simulink model "Microgrid_RL_Model"  (R2025b)
settings: Solver=ode23tb  StartTime=0.0  StopTime=12.0  MaxStep=0.01  RelTol=1e-8  AbsTol=1e-10
settings Model: Creator=ogare  LastModifiedBy=ogare

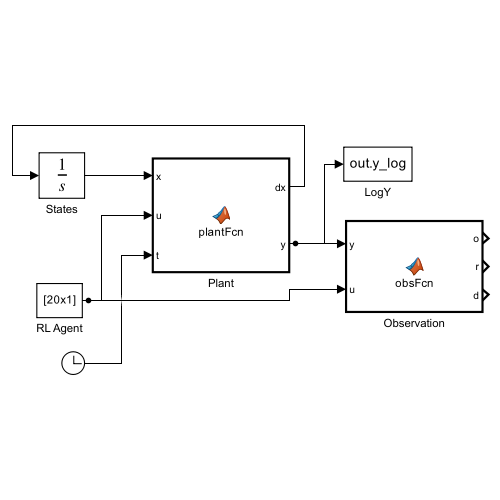
[thumbnail: Simulink's stored preview of the top-level diagram]
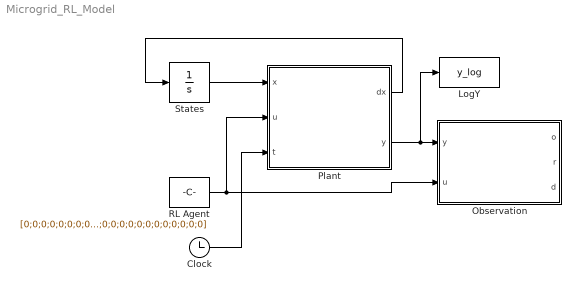
== system Microgrid_RL_Model ==
  Clock : Clock
  LogY : ToWorkspace  VariableName=y_log  SaveFormat=Structure With Time  SampleTime=0.01
  Observation : MATLAB Function  TreatAsAtomicUnit=on
  Plant : MATLAB Function  TreatAsAtomicUnit=on
  RL Agent : Constant  Value=[0;0;0;0;0;0;0;0;0;0;0;0;0;0;0;0;0;0;0;0]
  States : Integrator  InitialCondition=[0;0;0;0;0;0;0;0;0;0;0.65;0.65;0.65;0.65;0.65;0.65;0.65;0.65;0.65;0.65;0.28;0.28;0.28;0.28;0.28;0.28;0.28;0.28;0.28;0.28;0;0;0;0;0;0;0;0;0;0;0;0;0;0;0;0;0;0;0;0;1;1;1;1;1;1;1;1;1;1]
  wires:
  States/1 -> Plant/1(x)
  Clock/1 -> Plant/3(t)
  RL Agent/1 -> Observation/2(u), Plant/2(u)
  Plant/1(dx) -> States/1
  Plant/2(y) -> LogY/1, Observation/1(y)

== matlab function Microgrid_RL_Model/Observation ==
  data: y input; u input; o output; r output; d output
function [o, r, d] = obsFcn(y, u)
%#codegen
n = 10;
p = mg_params();
V = y(1:n); f = y(n+1:2*n); P = y(2*n+1:3*n); Q = y(3*n+1:4*n);
xi = y(5*n+1:6*n); ze = y(6*n+1:7*n);
xi_rx = y(7*n+1:8*n); ze_rx = y(8*n+1:9*n);
deg = max(sum(p.adj,1).', 1);
inn_xi = (p.adj.'*xi - sum(p.adj,1).'.*xi_rx) ./ deg;
inn_ze = (p.adj.'*ze - sum(p.adj,1).'.*ze_rx) ./ deg;
o = [V-1.0; (f-50)*10; P-0.5; Q-0.2; xi/p.xi_lim; ze/p.zeta_lim; ...
     inn_xi/p.xi_lim; inn_ze/p.zeta_lim];
% Reward mirrors mgxrl/envs/resilient_env.py. The control cost is
% CONNECTIVITY LOSS mean(1 - trust), not mean(u.^2): under trust weights
% every u >= 0 is full trust and costs nothing, so charging u.^2 taxes a
% harmless half of the action space and understate real isolations.
% The old 0.10 coefficient is also the value that made saturation free and
% collapsed the first policy; w_action is 1.0.
refs = [5.0e-4; 1.8e-3; 6.0e-3; 1.8e-1];
wts  = [3.0; 2.0; 1.5; 1.0];
met  = [sqrt(mean((f-50).^2)); sqrt(mean((V-1).^2)); ...
        std(P)/(mean(abs(P))+1e-9); std(Q)/(mean(abs(Q))+1e-9)];
trust = min(max(1 + u, 0), 1);
iso = mean(1 - trust);
viol = 50.0 * (any(V < 0.95) || any(V > 1.05));
r = 9.0 - sum(wts .* log1p((met./refs).^2)) - 1.0*iso - 6.0*(iso > 0.5) - viol;
d = any(V < 0.5) || any(V > 1.5) || any(abs(f-50) > 0.5);
end

== matlab function Microgrid_RL_Model/Plant ==
  data: x input; dx output; u input; y output; t input
function [dx, y] = plantFcn(x, u, t)
%#codegen
p   = mg_params();
atk = getAttackConfig();
[dx, y] = mg_dynamics(t, x, u, p, atk);
end
